simulink model "KMHE_UNEJ_TD10_ONLY"  (R2025b)
settings: Solver=FixedStepDiscrete  StartTime=0.0  StopTime=1500.05  FixedStep=0.05  RelTol=1e-3
model workspace (MAT data in the model file):
  KMHE_CFG.root = 'C:\Users\Hype G12\Documents\Kuliah\Semester 4\Rakata\urban\RAKATA_KMHE_MATLAB_SIMULINK\RAKATA_TD10_ONLY'
  KMHE_CFG.source = 'C:\Users\Hype G12\Documents\Kuliah\Semester 4\Rakata\urban\RAKATA_KMHE_MATLAB_SIMULINK\RAKATA_TD10_ONLY\data\TD10_latest.xlsx'
  KMHE_CFG.output = 'C:\Users\Hype G12\Documents\Kuliah\Semester 4\Rakata\urban\RAKATA_KMHE_MATLAB_SIMULINK\RAKATA_TD10_ONLY\results'
  KMHE_CFG.mass_kg = 141
  KMHE_CFG.ratio = 11
  KMHE_CFG.training_mass_kg = 141
  KMHE_CFG.voltage_V = 54
  KMHE_CFG.dt = 0.05
  KMHE_CFG.laps = 6
  KMHE_CFG.limit_s = 1500
  KMHE_CFG.length_m = 1600
  KMHE_CFG.stop_m = 665
  KMHE_CFG.hold_s = 3
  KMHE_CFG.brake_mps2 = 0.65
  KMHE_CFG.lateral_mps2 = 1.5
  KMHE_CFG.corner_cap_floor_kmh = 20
  KMHE_CFG.max_speed_kmh = 35.25
  KMHE_CFG.grade_scale = 1
  KMHE_CFG.throttle_tau_s = 0.3
  KMHE_CFG.power_tau_s = 2
  KMHE_CFG.no_load_kmh = 35.7
  KMHE_CFG.q_exponent = 2
  KMHE_CFG.training_length_m = 1440
  KMHE_CFG.train_laps = [1 4 5 7 8 10 13]
  KMHE_CFG.test_laps = [3 6 12 15]
  KMHE_CFG.max_gap_s = 0.5
  KMHE_CFG.seed = 10
  KMHE_CFG.search_trials = 300
  KMHE_CFG.max_time_error_s = 10
  KMHE_CFG.max_speed_rmse_kmh = 3
  KMHE_CFG.max_energy_mae_Wh = 0.5
  KMHE_CFG.allow_unvalidated_search = 1
  KMHE_CFG.zones = [0  100  100  35; 390  455  100  22; 665  895  100  35; 1185  1390  100  35]
  KMHE_CFG.launch_after_stop_until_m = 760
  KMHE_CFG.launch_after_stop_pct = 45
  KMHE_CFG.launch_after_stop_kmh = 20
  KMHE_MODEL.acceleration_coefficients = [-0.0548787164187; 0.000238986749526; 3; 0.982209992053; 0.421204060721; 0.639393718273; 0.397020167077; 0.158608302568; -0.0240041887518; 0.00878974138431; 0.0170124446384; -0.00556024273981; 0.00615931199275; 0.0107595440688; 0.045225567005; 0.0342900261113]
  KMHE_MODEL.power_coefficients = [828.739364706; 620.796240552; 723.530534688; 714.465952516; 811.141136217; 250.203765699]
  KMHE_MODEL.nodes = [0 7 14 21 28 36]
  KMHE_MODEL.idle_W = 6.96063529412
  KMHE_MODEL.voltage_V = 54
  KMHE_MODEL.power_tau_s = 2
  KMHE_MODEL.throttle_tau_s = 0.3
  KMHE_MODEL.trained_laps = [1 4 5 7 8 10 13]
  KMHE_MODEL.heldout_laps = [3 6 12 15]
  KMHE_MODEL.mass_kg = 141
  KMHE_MODEL.ratio = 11
  KMHE_MODEL.source = 'TD10_latest.xlsx only'
  KMHE_MODEL.coefficient_bounds_hit = 3
  KMHE_POLICY = [0  250  100  32.6871157331; 360  505  75  26; 665  1025  100  31.6617621885; 1185  1280  95  29.4160914119]
  KMHE_TRACK.s = [0; 5; 10; 15; 20; 25; 30; 35; 40; 45; 50; 55; 60; 65; 70; 75; 80; 85; 90; 95; 100; 105; 110; 115; 120; 125; 130; 135; 140; 145; 150; 155; 160; 165; 170; 175; 180; 185; 190; 195; 200; 205; 210; 215; 220; 225; 230; 235; 240; 245; 250; 255; 260; 265; 270; 275; 280; 285; 290; 295; 300; 305; 310; 315; 320; 325; 330; 335; 340; 345; 350; 355; 360; 365; 370; 375; 380; 385; 390; 395; 400; 405; 410; 415; 420; 425; 430; 435; 440; 445; 450; 455; 460; 465; 470; 475; 480; 485; 490; 495; 500; 505; 510; 515; 520; 525; 530; 535; 540; 545; 550; 555; 560; 565; 570; 575; 580; 585; 590; 595; 600; 605; 610; 615; 620; 625; 630; 635; 640; 645; 650; 655; 660; 665; 670; 675; 680; 685; 690; 695; 700; 705; 710; 715; 720; 725; 730; 735; 740; 745; 750; 755; 760; 765; 770; 775; 780; 785; 790; 795; 800; 805; 810; 815; 820; 825; 830; 835; 840; 845; 850; 855; 860; 865; 870; 875; 880; 885; 890; 895; 900; 905; 910; 915; 920; 925; 930; 935; 940; 945; 950; 955; 960; 965; 970; 975; 980; 985; 990; 995; 1000; 1005; 1010; 1015; 1020; 1025; 1030; 1035; 1040; 1045; 1050; 1055; 1060; 1065; 1070; 1075; 1080; 1085; 1090; 1095; 1100; 1105; 1110; 1115; 1120; 1125; 1130; 1135; 1140; 1145; 1150; 1155; 1160; 1165; 1170; 1175; 1180; 1185; 1190; 1195; 1200; 1205; 1210; 1215; 1220; 1225; 1230; 1235; 1240; 1245; 1250; 1255; 1260; 1265; 1270; 1275; 1280; 1285; 1290; 1295; 1300; 1305; 1310; 1315; 1320; 1325; 1330; 1335; 1340; 1345; 1350; 1355; 1360; 1365; 1370; 1375; 1380; 1385; 1390; 1395; 1400; 1405; 1410; 1415; 1420; 1425; 1430; 1435; 1440; 1445; 1450; 1455; 1460; 1465; 1470; 1475; 1480; 1485; 1490; 1495; 1500; 1505; 1510; 1515; 1520; 1525; 1530; 1535; 1540; 1545; 1550; 1555; 1560; 1565; 1570; 1575; 1580; 1585; 1590; 1595; 1600]
  KMHE_TRACK.lat = [-8.1646108 -8.16458811419 -8.16456542837 -8.16454274256 -8.16452005674 -8.16449737093 -8.16447468512 -8.1644519993 -8.16442931349 -8.16440659647 -8.1643828131 -8.16435722047 ... (321 elements, 321x1)]
  KMHE_TRACK.lng = [113.7152654 113.715303933 113.715342467 113.715381 113.715419533 113.715458067 113.7154966 113.715535133 113.715573667 113.715612181 113.715650026 113.715686647 ... (321 elements, 321x1)]
  KMHE_TRACK.raw_elevation = [100.902984262 100.862868238 100.805651604 100.735331475 100.655904966 100.557622969 100.43485271 100.297765802 100.156533861 100.004200624 99.8371846621 99.6707198385 ... (321 elements, 321x1)]
  KMHE_TRACK.raw_grade = [-0.00802320485114 -0.00973326582083 -0.0127536762748 -0.0149746637578 -0.0177708505565 -0.0221052256348 -0.0259857167218 -0.0278318848697 -0.0293565177907 -0.0319349199078 -0.0333480785747 -0.0317144644347 ... (321 elements, 321x1)]
  KMHE_TRACK.net_grade_correction = -0.00269669456332
  KMHE_TRACK.grade = [-0.00532651028783 -0.00703657125751 -0.0100569817114 -0.0122779691945 -0.0150741559932 -0.0194085310715 -0.0232890221585 -0.0251351903064 -0.0266598232274 -0.0292382253444 -0.0306513840114 -0.0290177698714 ... (321 elements, 321x1)]
  KMHE_TRACK.elevation = [100.902984262 100.872076558 100.829342676 100.773505298 100.705124985 100.618918268 100.512174385 100.391113854 100.26162632 100.121881198 99.9721571749 99.8229842902 ... (321 elements, 321x1)]
  KMHE_TRACK.raw_lat = [-8.1646108 -8.16458811419 -8.16456542837 -8.16454274256 -8.16452005674 -8.16449737093 -8.16447468512 -8.1644519993 -8.16442931349 -8.16440659647 -8.1643828131 -8.16435722047 ... (321 elements, 321x1)]
  KMHE_TRACK.raw_lng = [113.7152654 113.715303933 113.715342467 113.715381 113.715419533 113.715458067 113.7154966 113.715535133 113.715573667 113.715612181 113.715650026 113.715686647 ... (321 elements, 321x1)]
  KMHE_TRACK.status = 'Estimated closure: final 50 m geometry blended; mean grade removed'
  KMHE_TRACK.speed_cap = [35.25 35.25 35.25 35.25 35.25 35.25 35.25 35.25 35.25 35.25 35.25 35.25 ... (321 elements, 321x1)]
  KMHE_TRACK.geometry_speed_cap = [35.25 35.25 35.25 35.25 35.25 35.25 35.25 35.25 35.25 35.25 35.25 35.25 ... (321 elements, 321x1)]
  KMHE_TRACK.markers(1).n = 1
  KMHE_TRACK.markers(1).s = 0
  KMHE_TRACK.markers(1).lat = -8.1646108
  KMHE_TRACK.markers(1).lng = 113.7152654
  KMHE_TRACK.markers(1).method = 'schematic affine projection onto reconstructed OSM route'
  KMHE_TRACK.markers(2).n = 2
  KMHE_TRACK.markers(2).s = 100
  KMHE_TRACK.markers(2).lat = -8.16418621105
  KMHE_TRACK.markers(2).lng = 113.716038591
  KMHE_TRACK.markers(2).method = 'schematic affine projection onto reconstructed OSM route'
  KMHE_TRACK.markers(3).n = 3
  KMHE_TRACK.markers(3).s = 165
  KMHE_TRACK.markers(3).lat = -8.16436156757
  KMHE_TRACK.markers(3).lng = 113.716592678
  KMHE_TRACK.markers(3).method = 'schematic affine projection onto reconstructed OSM route'
  KMHE_TRACK.markers(4).n = 4
  KMHE_TRACK.markers(4).s = 240
  KMHE_TRACK.markers(4).lat = -8.16391116181
  KMHE_TRACK.markers(4).lng = 113.716929487
  KMHE_TRACK.markers(4).method = 'schematic affine projection onto reconstructed OSM route'
  KMHE_TRACK.markers(5).n = 5
  KMHE_TRACK.markers(5).s = 305
  KMHE_TRACK.markers(5).lat = -8.16394096932
  KMHE_TRACK.markers(5).lng = 113.717501104
  KMHE_TRACK.markers(5).method = 'schematic affine projection onto reconstructed OSM route'
  KMHE_TRACK.markers(6).n = 6
  KMHE_TRACK.markers(6).s = 390
  KMHE_TRACK.markers(6).lat = -8.164682379
  KMHE_TRACK.markers(6).lng = 113.71747498
  KMHE_TRACK.markers(6).method = 'schematic affine projection onto reconstructed OSM route'
  KMHE_TRACK.markers(7).n = 7
  KMHE_TRACK.markers(7).s = 455
  KMHE_TRACK.markers(7).lat = -8.16489438669
  KMHE_TRACK.markers(7).lng = 113.718016825
  KMHE_TRACK.markers(7).method = 'schematic affine projection onto reconstructed OSM route'
  KMHE_TRACK.markers(8).n = 8
  KMHE_TRACK.markers(8).s = 580
  KMHE_TRACK.markers(8).lat = -8.16532093748
  KMHE_TRACK.markers(8).lng = 113.719049822
  KMHE_TRACK.markers(8).method = 'schematic affine projection onto reconstructed OSM route'
  KMHE_TRACK.markers(9).n = 9
  KMHE_TRACK.markers(9).s = 665
  KMHE_TRACK.markers(9).lat = -8.16600538323
  KMHE_TRACK.markers(9).lng = 113.718741351
  KMHE_TRACK.markers(9).method = 'schematic affine projection onto reconstructed OSM route'
  KMHE_TRACK.markers(10).n = 10
  KMHE_TRACK.markers(10).s = 760
  KMHE_TRACK.markers(10).lat = -8.16676221849
  KMHE_TRACK.markers(10).lng = 113.718370147
  KMHE_TRACK.markers(10).method = 'schematic affine projection onto reconstructed OSM route'
  KMHE_TRACK.markers(11).n = 11
  KMHE_TRACK.markers(11).s = 890
  KMHE_TRACK.markers(11).lat = -8.16635878727
  KMHE_TRACK.markers(11).lng = 113.71728393
  KMHE_TRACK.markers(11).method = 'schematic affine projection onto reconstructed OSM route'
  KMHE_TRACK.markers(12).n = 12
  KMHE_TRACK.markers(12).s = 995
  KMHE_TRACK.markers(12).lat = -8.1660193139
  KMHE_TRACK.markers(12).lng = 113.716407163
  KMHE_TRACK.markers(12).method = 'schematic affine projection onto reconstructed OSM route'
  KMHE_TRACK.markers(13).n = 13
  KMHE_TRACK.markers(13).s = 1180
  KMHE_TRACK.markers(13).lat = -8.16750414076
  KMHE_TRACK.markers(13).lng = 113.715729754
  KMHE_TRACK.markers(13).method = 'schematic affine projection onto reconstructed OSM route'
  KMHE_TRACK.markers(14).n = 14
  KMHE_TRACK.markers(14).s = 1345
  KMHE_TRACK.markers(14).lat = -8.16675327179
  KMHE_TRACK.markers(14).lng = 113.71450042
  KMHE_TRACK.markers(14).method = 'schematic affine projection onto reconstructed OSM route'
  KMHE_TRACK.markers(15).n = 15
  KMHE_TRACK.markers(15).s = 1485
  KMHE_TRACK.markers(15).lat = -8.16555323429
  KMHE_TRACK.markers(15).lng = 113.714639471
  KMHE_TRACK.markers(15).method = 'schematic affine projection onto reconstructed OSM route'
  KMHE_TRACK.markers(16).n = 16
  KMHE_TRACK.markers(16).s = 1550
  KMHE_TRACK.markers(16).lat = -8.16527293642
  KMHE_TRACK.markers(16).lng = 113.715146396
  KMHE_TRACK.markers(16).method = 'schematic affine projection onto reconstructed OSM route'
  KMHE_TRACK.markers(17).n = 17
  KMHE_TRACK.markers(17).s = 1600
  KMHE_TRACK.markers(17).lat = -8.16491375398
  KMHE_TRACK.markers(17).lng = 113.715239432
  KMHE_TRACK.markers(17).method = 'schematic affine projection onto reconstructed OSM route'
  KMHE_TRACK.markers(18).n = 18
  KMHE_TRACK.markers(18).s = 1580
  KMHE_TRACK.markers(18).lat = -8.16508806747
  KMHE_TRACK.markers(18).lng = 113.715273345
  KMHE_TRACK.markers(18).method = 'schematic affine projection onto reconstructed OSM route'
  manual_input = [0  0  0; 1  0  0; 4  100  0; 12  0  0; 1500  0  0]
settings Model: Creator=Hype G12  LastModifiedBy=Hype G12

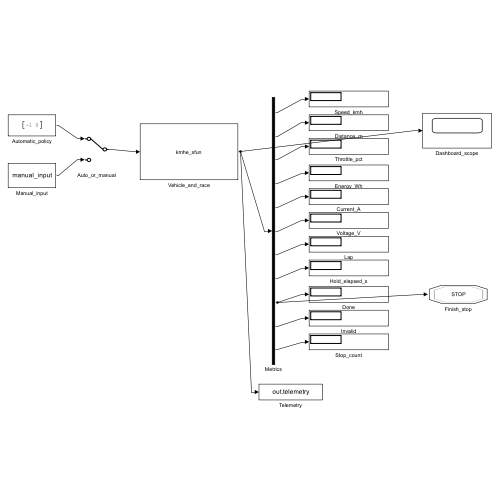
[thumbnail: Simulink's stored preview of the top-level diagram]
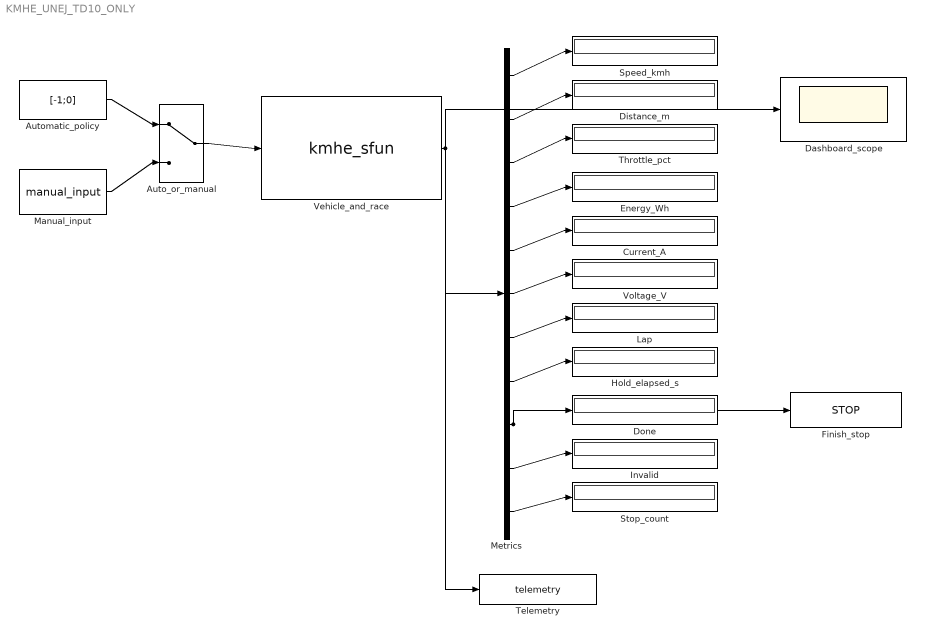
== system KMHE_UNEJ_TD10_ONLY ==
  Auto_or_manual : ManualSwitch
  Automatic_policy : Constant  Value=[-1;0]
  Current_A : Display
  Dashboard_scope : Scope
  Distance_m : Display
  Done : Display
  Energy_Wh : Display
  Finish_stop : Stop
  Hold_elapsed_s : Display
  Invalid : Display
  Lap : Display
  Manual_input : FromWorkspace  VariableName=manual_input  SampleTime=KMHE_CFG.dt  Interpolate=off  ZeroCross=off  OutputAfterFinalValue=Holding final value
  Metrics : Demux  Outputs=11
  Speed_kmh : Display
  Stop_count : Display
  Telemetry : ToWorkspace  VariableName=telemetry  SaveFormat=Timeseries  SampleTime=-1
  Throttle_pct : Display
  Vehicle_and_race : M-S-Function  FunctionName=kmhe_sfun  Parameters=KMHE_CFG,KMHE_MODEL,KMHE_TRACK,KMHE_POLICY
  Voltage_V : Display
  wires:
  Metrics/1 -> Speed_kmh/1
  Metrics/2 -> Distance_m/1
  Metrics/3 -> Throttle_pct/1
  Metrics/4 -> Energy_Wh/1
  Metrics/5 -> Current_A/1
  Metrics/6 -> Voltage_V/1
  Metrics/7 -> Lap/1
  Metrics/8 -> Hold_elapsed_s/1
  Metrics/9 -> Done/1, Finish_stop/1
  Metrics/10 -> Invalid/1
  Metrics/11 -> Stop_count/1
  Automatic_policy/1 -> Auto_or_manual/1
  Manual_input/1 -> Auto_or_manual/2
  Auto_or_manual/1 -> Vehicle_and_race/1
  Vehicle_and_race/1 -> Metrics/1, Telemetry/1, Dashboard_scope/1
